simulink model "FMS"  (R2018b)
settings: configuration reference "fms_config" (kept outside this file)
values from neighbouring files (symbols this model uses):
  FMS_EXPORT = Simulink.Parameter(FMS_EXPORT_VALUE)    [fms_model_init.m]
  FMS_PARAM = Simulink.Parameter(FMS_PARAM_VALUE)    [fms_model_init.m]
undefined symbols (not defined in the file or in its folder): actuator_cmd, ax_cmd, ay_cmd, az_cmd, cmd_mask, ControlMode, ctrl_mode, DiscIntNeverNeededParam, ext_state, FMS_Cmd, FMS_CONST, home, mode, p_cmd, phi_cmd, PilotMode, psi_rate_cmd, q_cmd, r_cmd, reset, state, status, theta_cmd, throttle_cmd, timestamp, u_cmd, v_cmd, VehicleState, VehicleStatus, VTOLState, w_cmd, wp_consume, wp_current
libraries: simulink x141, FMT_Model_Lib x120, hdlsllib x13
(part 1 of 12)
settings Model: Creator=jc  LastModifiedBy=zouji
settings ConfigSetRef: SourceLocation=Base Workspace

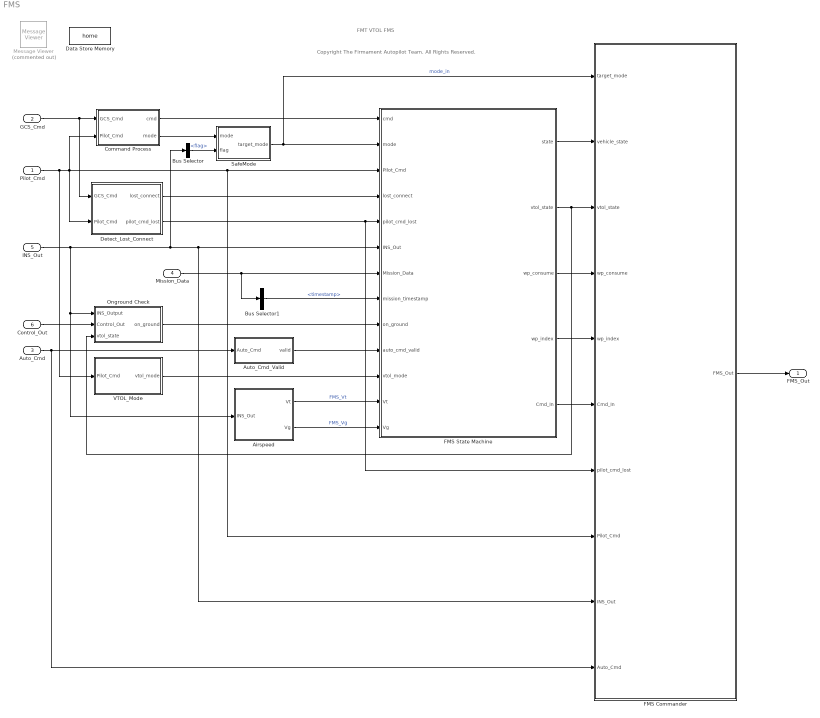
== system FMS ==
  note: Copyright The Firmament Autopilot Team. All Rights Reserved.
  note: FMT VTOL FMS
  Pilot_Cmd : Inport  OutDataTypeStr=Bus: Pilot_Cmd_Bus
  GCS_Cmd : Inport  Port=2  OutDataTypeStr=Bus: GCS_Cmd_Bus
  Auto_Cmd : Inport  Port=3  OutDataTypeStr=Bus: Auto_Cmd_Bus
  Mission_Data : Inport  Port=4  OutDataTypeStr=Bus: Mission_Data_Bus  BusOutputAsStruct=on
  INS_Out : Inport  Port=5  OutDataTypeStr=Bus: INS_Out_Bus
  Control_Out : Inport  Port=6  OutDataTypeStr=Bus: Control_Out_Bus
  Airspeed : Subsystem
  Auto_Cmd_Valid : Subsystem
  Bus Selector : BusSelector  OutputSignals=flag
  Bus Selector1 : BusSelector  OutputSignals=timestamp
  Command Process : Subsystem
  Data Store Memory : DataStoreMemory  DataStoreName=home  ReadBeforeWriteMsg=warning  WriteAfterWriteMsg=warning  WriteAfterReadMsg=warning  ShowAdditionalParam=off  OutDataTypeStr=single  Dimensions=4
  Detect_Lost_Connect : Subsystem
  FMS Commander : Subsystem  TreatAsAtomicUnit=on
  FMS State Machine : Stateflow chart  TreatAsAtomicUnit=on
  Message Viewer : MessageViewer  Commented=on  SavedRootId=#
  Onground Check : Subsystem
  SafeMode : Stateflow chart  TreatAsAtomicUnit=on
  VTOL_Mode : Subsystem
  FMS_Out : Outport  OutDataTypeStr=Bus: FMS_Out_Bus
  wires:
  Control_Out/1 -> Onground Check/2(Control_Out)
  Command Process/1(cmd) -> FMS State Machine/1(cmd)
  FMS State Machine/5(Cmd_In) -> FMS Commander/6(Cmd_In)
  Pilot_Cmd/1 -> VTOL_Mode/1(Pilot_Cmd), Detect_Lost_Connect/2(Pilot_Cmd), FMS Commander/8(Pilot_Cmd), FMS State Machine/3(Pilot_Cmd), Command Process/2(Pilot_Cmd)
  INS_Out/1 -> Airspeed/1(INS_Out), Onground Check/1(INS_Output), Bus Selector/1, FMS Commander/9(INS_Out), FMS State Machine/6(INS_Out)
  Command Process/2(mode) -> SafeMode/1(mode)
  FMS Commander/1(FMS_Out) -> FMS_Out/1
  Onground Check/1(on_ground) -> FMS State Machine/9(on_ground)
  Bus Selector/1 -> SafeMode/2(flag)  "<flag>"
  GCS_Cmd/1 -> Detect_Lost_Connect/1(GCS_Cmd), Command Process/1(GCS_Cmd)
  SafeMode/1(target_mode) -> FMS Commander/1(target_mode), FMS State Machine/2(mode)  "mode_in"
  FMS State Machine/1(state) -> FMS Commander/2(vehicle_state)
  Mission_Data/1 -> Bus Selector1/1, FMS State Machine/7(Mission_Data)
  FMS State Machine/3(wp_consume) -> FMS Commander/4(wp_consume)
  Bus Selector1/1 -> FMS State Machine/8(mission_timestamp)  "<timestamp>"
  FMS State Machine/4(wp_index) -> FMS Commander/5(wp_index)
  Auto_Cmd/1 -> Auto_Cmd_Valid/1(Auto_Cmd), FMS Commander/10(Auto_Cmd)
  Auto_Cmd_Valid/1(valid) -> FMS State Machine/10(auto_cmd_valid)
  Detect_Lost_Connect/1(lost_connect) -> FMS State Machine/4(lost_connect)
  Detect_Lost_Connect/2(pilot_cmd_lost) -> FMS State Machine/5(pilot_cmd_lost), FMS Commander/7(pilot_cmd_lost)
  Airspeed/2(Vg) -> FMS State Machine/13(Vg)  "FMS_Vg"
  Airspeed/1(Vt) -> FMS State Machine/12(Vt)  "FMS_Vt"
  VTOL_Mode/1(vtol_mode) -> FMS State Machine/11(vtol_mode)
  FMS State Machine/2(vtol_state) -> Onground Check/3(vtol_state), FMS Commander/3(vtol_state)

== system FMS/Airspeed ==
  note: If airspeed is invalid, use ground speed
  INS_Out : Inport
  Add : Sum
  Bitwise AND : simulink/Logic and Bit Operations/Bitwise Operator  logicop=AND  UseBitMask=on  BitMask=bin2dec('1000000000')  BitMaskRealWorld=Stored Integer
  Bus Selector1 : BusSelector  OutputSignals=vn,ve
  Bus Selector2 : BusSelector  OutputSignals=flag
  Bus Selector3 : BusSelector  OutputSignals=airspeed
  First Order LPF1 : FMT_Model_Lib/Filter/First Order LPF  fc=20
      settings: SourceProductName=FMT Toolbox
  First Order LPF3 : FMT_Model_Lib/Filter/First Order LPF  fc=10
      settings: SourceProductName=FMT Toolbox
  Fly_Direction : Subsystem
  Fly_Speed : Subsystem
  Multiply : Product
  Saturation1 : Saturate  UpperLimit=100  LowerLimit=0.1
  Sqrt : Sqrt  SaturateOnIntegerOverflow=on
  Square2 : Math  Operator=square  SaturateOnIntegerOverflow=on
  Square3 : Math  Operator=square  SaturateOnIntegerOverflow=on
  Switch : Switch  Criteria=u2 > Threshold
  Vt : Outport
  Vg : Outport  Port=2
  wires:
  Square3/1 -> Add/2
  Sqrt/1 -> Multiply/2
  Bus Selector1/1 -> Square2/1  "<vn>"
  Fly_Direction/1(sign) -> Multiply/1
  Add/1 -> Sqrt/1
  Square2/1 -> Add/1
  Bus Selector1/2 -> Square3/1  "<ve>"
  Multiply/1 -> First Order LPF1/1  "Vg"
  Switch/1 -> Saturation1/1
  Saturation1/1 -> First Order LPF3/1
  INS_Out/1 -> Fly_Direction/1(INS_Out), Bus Selector1/1, Fly_Speed/1(INS_Out), Bus Selector2/1, Bus Selector3/1
  Bitwise AND/1 -> Switch/2
  Bus Selector2/1 -> Bitwise AND/1  "<flag>"
  Bus Selector3/1 -> Switch/1  "<airspeed>"
  First Order LPF1/1 -> Vg/1
  First Order LPF3/1 -> Vt/1
  Fly_Speed/1(speed) -> Switch/3

== system FMS/Auto_Cmd_Valid ==
  Auto_Cmd : Inport
  Bus Selector1 : BusSelector  OutputSignals=frame
  Bus Selector2 : BusSelector  OutputSignals=timestamp
  Compare To Constant4 : simulink/Logic and Bit Operations/Compare To Constant  relop=<  const=1000  OutDataTypeStr=boolean
  Constant : Constant  Value=FMS_EXPORT.period  OutDataTypeStr=single
  Detect Change : simulink/Logic and Bit Operations/Detect Change  vinit=0  OutDataTypeStr=boolean
  Discrete-Time Integrator : DiscreteIntegrator  IntegratorMethod=Accumulation: Forward Euler  ExternalReset=sampled level  SampleTime=-1  OutDataTypeStr=uint32  SaturateOnIntegerOverflow=on  ICPrevOutput=DiscIntNeverNeededParam  ICPrevScaledInput=DiscIntNeverNeededParam
  Ever_Valid : Subsystem
  Interval Test : simulink/Logic and Bit Operations/Interval Test  IntervalClosedRight=on  uplimit=2  IntervalClosedLeft=on  lowlimit=0  OutDataTypeStr=boolean
  Logical Operator : Logic  Inputs=3  AllPortsSameDT=off  OutDataTypeStr=boolean
  valid : Outport
  wires:
  Constant/1 -> Discrete-Time Integrator/1
  Detect Change/1 -> Ever_Valid/1(in), Discrete-Time Integrator/2
  Discrete-Time Integrator/1 -> Compare To Constant4/1
  Auto_Cmd/1 -> Bus Selector1/1, Bus Selector2/1
  Compare To Constant4/1 -> Logical Operator/1
  Ever_Valid/1(out) -> Logical Operator/2
  Logical Operator/1 -> valid/1
  Bus Selector2/1 -> Detect Change/1  "<timestamp>"
  Bus Selector1/1 -> Interval Test/1  "<frame>"
  Interval Test/1 -> Logical Operator/3

== system FMS/Command Process ==
  GCS_Cmd : Inport
  Pilot_Cmd : Inport  Port=2
  Check Valid : Subsystem
  Command PreProcess : Subsystem
  Mode PreProcess : Subsystem
  cmd : Outport
  mode : Outport  Port=2
  wires:
  GCS_Cmd/1 -> Mode PreProcess/2(GCS_Cmd), Command PreProcess/1(gcs_cmd)
  Pilot_Cmd/1 -> Command PreProcess/2(pilot_cmd), Check Valid/1(Pilot_Cmd), Mode PreProcess/3(Pilot_Cmd)
  Command PreProcess/1(cmd_1) -> cmd/1  "fms_cmd"
  Check Valid/1(pilot_cmd_valid) -> Mode PreProcess/1(pilot_cmd_valid)
  Mode PreProcess/1(mode) -> mode/1  "fms_mode"

== system FMS/Detect_Lost_Connect ==
  GCS_Cmd : Inport
  Pilot_Cmd : Inport  Port=2
  Bus Selector : BusSelector  OutputSignals=timestamp
  Bus Selector1 : BusSelector  OutputSignals=timestamp
  Constant : Constant  Value=FMS_CONST.dt  OutDataTypeStr=single
  Constant1 : Constant  Value=FMS_PARAM.LOST_RETURN_EN
  Detect Change : simulink/Logic and Bit Operations/Detect Change  vinit=0  OutDataTypeStr=boolean
  Detect Change1 : simulink/Logic and Bit Operations/Detect Change  vinit=0  OutDataTypeStr=boolean
  Discrete-Time Integrator : DiscreteIntegrator  IntegratorMethod=Accumulation: Forward Euler  ExternalReset=sampled level  SampleTime=-1  OutDataTypeStr=single  SaturateOnIntegerOverflow=on  LimitOutput=on  UpperSaturationLimit=65535  LowerSaturationLimit=0  ICPrevOutput=DiscIntNeverNeededParam  ICPrevScaledInput=DiscIntNeverNeededParam
  Discrete-Time Integrator1 : DiscreteIntegrator  IntegratorMethod=Accumulation: Forward Euler  ExternalReset=sampled level  SampleTime=-1  OutDataTypeStr=single  SaturateOnIntegerOverflow=on  LimitOutput=on  UpperSaturationLimit=65535  LowerSaturationLimit=0  ICPrevOutput=DiscIntNeverNeededParam  ICPrevScaledInput=DiscIntNeverNeededParam
  Logical Operator : Logic  Operator=OR  Inputs=3  AllPortsSameDT=off  OutDataTypeStr=boolean
  Logical Operator1 : Logic  Operator=NOT  AllPortsSameDT=off  OutDataTypeStr=boolean
  Logical Operator2 : Logic  AllPortsSameDT=off  OutDataTypeStr=boolean
  timeout1_s : simulink/Logic and Bit Operations/Compare To Constant  relop=>=  const=FMS_PARAM.LOST_RETURN_TIME  OutDataTypeStr=boolean
  timeout2_s : simulink/Logic and Bit Operations/Compare To Constant  relop=>=  const=1  OutDataTypeStr=boolean
  lost_connect : Outport
  pilot_cmd_lost : Outport  Port=2
  wires:
  Constant/1 -> Discrete-Time Integrator1/1, Discrete-Time Integrator/1
  Discrete-Time Integrator/1 -> timeout1_s/1
  GCS_Cmd/1 -> Bus Selector/1
  Pilot_Cmd/1 -> Bus Selector1/1
  Bus Selector/1 -> Detect Change/1  "<timestamp>"
  Bus Selector1/1 -> Detect Change1/1  "<timestamp>"
  Detect Change/1 -> Logical Operator/1
  Detect Change1/1 -> Discrete-Time Integrator1/2, Logical Operator/2
  Constant1/1 -> Logical Operator2/2, Logical Operator1/1
  Logical Operator1/1 -> Logical Operator/3
  Logical Operator/1 -> Discrete-Time Integrator/2
  Logical Operator2/1 -> lost_connect/1
  timeout1_s/1 -> Logical Operator2/1
  Discrete-Time Integrator1/1 -> timeout2_s/1
  timeout2_s/1 -> pilot_cmd_lost/1

== system FMS/FMS Commander ==
  target_mode : Inport
  vehicle_state : Inport  Port=2
  vtol_state : Inport  Port=3
  wp_consume : Inport  Port=4
  wp_index : Inport  Port=5
  Cmd_In : Inport  Port=6
  pilot_cmd_lost : Inport  Port=7
  Pilot_Cmd : Inport  Port=8
  INS_Out : Inport  Port=9
  Auto_Cmd : Inport  Port=10
  Commander : Subsystem
  FMS_Input : Subsystem  TreatAsAtomicUnit=on
  FMS_Out : Outport
  wires:
  target_mode/1 -> Commander/1(target_mode)
  FMS_Input/1(FMS_In) -> Commander/2(FMS_In)  "FMS_In"
  Commander/1(FMS_Out) -> FMS_Out/1
  vehicle_state/1 -> FMS_Input/1(state)
  wp_consume/1 -> FMS_Input/3(wp_consume)
  wp_index/1 -> FMS_Input/4(wp_index)
  Cmd_In/1 -> FMS_Input/5(Cmd_In)
  Pilot_Cmd/1 -> FMS_Input/7(Pilot_Cmd)
  INS_Out/1 -> FMS_Input/8(INS_Out)
  Auto_Cmd/1 -> FMS_Input/9(Auto_Cmd)
  pilot_cmd_lost/1 -> FMS_Input/6(pilot_cmd_lost)
  vtol_state/1 -> FMS_Input/2(vtol_state)

== system FMS/FMS State Machine/VTOL_State.EndStall ==
  Airspeed : Inport  OutDataTypeStr=single  PortDimensions=1
  f : TriggerPort  TriggerType=function-call  VariantControl=(inherit)  StatesWhenEnabling=reset
      settings: CopyFcn=Stateflow.SLINSF.SimulinkMan.removeBlockPreDeleteFcn  PreDeleteFcn=Stateflow.SLINSF.SimulinkMan.unsafePredeleteFcn
  Constant1 : Constant  Value=FMS_PARAM.FW_SPEED_MIN
  Relational Operator1 : RelationalOperator  OutDataTypeStr=boolean  RndMeth=Simplest
  res : Outport
  wires:
  Airspeed/1 -> Relational Operator1/1
  Constant1/1 -> Relational Operator1/2
  Relational Operator1/1 -> res/1

== system FMS/FMS State Machine/VTOL_State.ForwardTransCplt ==
  Airspeed : Inport  OutDataTypeStr=single  PortDimensions=1
  f : TriggerPort  TriggerType=function-call  VariantControl=(inherit)  StatesWhenEnabling=reset
      settings: CopyFcn=Stateflow.SLINSF.SimulinkMan.removeBlockPreDeleteFcn  PreDeleteFcn=Stateflow.SLINSF.SimulinkMan.unsafePredeleteFcn
  Constant : Constant  Value=FMS_PARAM.FW_SPEED_MIN
  Relational Operator : RelationalOperator  OutDataTypeStr=boolean  RndMeth=Simplest
  cplt : Outport
  wires:
  Airspeed/1 -> Relational Operator/1
  Constant/1 -> Relational Operator/2
  Relational Operator/1 -> cplt/1

== system FMS/FMS State Machine/VTOL_State.IsPosValid ==
  flag : Inport  OutDataTypeStr=uint32  PortDimensions=1
  f : TriggerPort  TriggerType=function-call  VariantControl=(inherit)  StatesWhenEnabling=reset
      settings: CopyFcn=Stateflow.SLINSF.SimulinkMan.removeBlockPreDeleteFcn  PreDeleteFcn=Stateflow.SLINSF.SimulinkMan.unsafePredeleteFcn
  Bitwise AND : simulink/Logic and Bit Operations/Bitwise Operator  logicop=AND  UseBitMask=on  BitMask=bin2dec('11010100')  BitMaskRealWorld=Stored Integer
  Compare To Constant : simulink/Logic and Bit Operations/Compare To Constant  relop===  const=bin2dec('11010100')  OutDataTypeStr=boolean
  valid : Outport
  wires:
  flag/1 -> Bitwise AND/1
  Bitwise AND/1 -> Compare To Constant/1
  Compare To Constant/1 -> valid/1

== system FMS/FMS State Machine/VTOL_State.IsStall ==
  Airspeed : Inport  OutDataTypeStr=single  PortDimensions=1
  f : TriggerPort  TriggerType=function-call  VariantControl=(inherit)  StatesWhenEnabling=reset
      settings: CopyFcn=Stateflow.SLINSF.SimulinkMan.removeBlockPreDeleteFcn  PreDeleteFcn=Stateflow.SLINSF.SimulinkMan.unsafePredeleteFcn
  Constant1 : Constant  Value=FMS_PARAM.FW_STALL_SPEED
  Relational Operator1 : RelationalOperator  Operator=<=  OutDataTypeStr=boolean  RndMeth=Simplest
  res : Outport
  wires:
  Airspeed/1 -> Relational Operator1/1
  Constant1/1 -> Relational Operator1/2
  Relational Operator1/1 -> res/1

== system FMS/FMS State Machine/Vehicle.AcceptRadius ==
  state : Inport  OutDataTypeStr=Enum: VTOLState  PortDimensions=1
  f : TriggerPort  TriggerType=function-call  VariantControl=(inherit)  StatesWhenEnabling=reset
      settings: CopyFcn=Stateflow.SLINSF.SimulinkMan.removeBlockPreDeleteFcn  PreDeleteFcn=Stateflow.SLINSF.SimulinkMan.unsafePredeleteFcn
  Compare To Constant : simulink/Logic and Bit Operations/Compare To Constant  relop===  const=VTOLState.Multicopter  OutDataTypeStr=boolean
  FW_ACCEPT_R : Constant  Value=FMS_PARAM.FW_ACCEPT_R
  MC_ACCEPT_R : Constant  Value=FMS_PARAM.MC_ACCEPT_R
  Switch : Switch  Criteria=u2 > Threshold
  radius : Outport
  wires:
  Compare To Constant/1 -> Switch/2
  FW_ACCEPT_R/1 -> Switch/3
  MC_ACCEPT_R/1 -> Switch/1
  Switch/1 -> radius/1
  state/1 -> Compare To Constant/1

== system FMS/FMS State Machine/Vehicle.Arm.Auto.Mission.LLA2FLAT ==
  lla : Inport  OutDataTypeStr=double  PortDimensions=[1 3]
  llo : Inport  Port=2  OutDataTypeStr=double  Unit=deg  PortDimensions=[1 2]
  href : Inport  Port=3  OutDataTypeStr=double  Unit=m  PortDimensions=1
  psio : Inport  Port=4  OutDataTypeStr=double  Unit=deg  PortDimensions=1
  f : TriggerPort  TriggerType=function-call  VariantControl=(inherit)
      settings: CopyFcn=Stateflow.SLINSF.SimulinkMan.removeBlockPreDeleteFcn  PreDeleteFcn=Stateflow.SLINSF.SimulinkMan.unsafePredeleteFcn
  Data Type Conversion : DataTypeConversion  OutDataTypeStr=single
  LLA2FLAT : FMT_Model_Lib/Transformation/LLA2FLAT
      settings: SourceProductName=FMT Toolbox
  Signal Conversion : SignalConversion  OverrideOpt=off
  pos : Outport
  wires:
  LLA2FLAT/1 -> Signal Conversion/1
  lla/1 -> LLA2FLAT/1
  llo/1 -> LLA2FLAT/2
  href/1 -> LLA2FLAT/3
  psio/1 -> LLA2FLAT/4
  Signal Conversion/1 -> Data Type Conversion/1
  Data Type Conversion/1 -> pos/1

== system FMS/FMS State Machine/Vehicle.HeadingErr ==
  psi_cmd : Inport  OutDataTypeStr=single  PortDimensions=1
  psi_est : Inport  Port=2  OutDataTypeStr=single  Unit=deg  PortDimensions=1
  f : TriggerPort  TriggerType=function-call  VariantControl=(inherit)
      settings: CopyFcn=Stateflow.SLINSF.SimulinkMan.removeBlockPreDeleteFcn  PreDeleteFcn=Stateflow.SLINSF.SimulinkMan.unsafePredeleteFcn
  Sum : Sum  Inputs=|+-
  psi_saturation : Subsystem
  err : Outport
  wires:
  psi_saturation/1(psi_rad) -> err/1
  psi_est/1 -> Sum/2
  psi_cmd/1 -> Sum/1
  Sum/1 -> psi_saturation/1(psi_in)

== system FMS/FMS State Machine/Vehicle.PrepTakeoff ==
  xy_R : Inport  OutDataTypeStr=single  PortDimensions=2
  f : TriggerPort  TriggerType=function-call  VariantControl=(inherit)  StatesWhenEnabling=reset
      settings: CopyFcn=Stateflow.SLINSF.SimulinkMan.removeBlockPreDeleteFcn  PreDeleteFcn=Stateflow.SLINSF.SimulinkMan.unsafePredeleteFcn
  Constant : Constant  Value=FMS_PARAM.TAKEOFF_H
  Mux : Mux  Inputs=2
  Reshape : Reshape  OutputDimensionality=Column vector (2-D)
  sp_takeoff : Outport
  wires:
  Reshape/1 -> sp_takeoff/1
  xy_R/1 -> Mux/1
  Mux/1 -> Reshape/1
  Constant/1 -> Mux/2

== system FMS/FMS State Machine/Vehicle.StickMoved ==
  stick_val : Inport  OutDataTypeStr=double  PortDimensions=4
  pilot_cmd : Inport  Port=2  OutDataTypeStr=Bus: Pilot_Cmd_Bus  PortDimensions=1
  f : TriggerPort  TriggerType=function-call  VariantControl=(inherit)
      settings: CopyFcn=Stateflow.SLINSF.SimulinkMan.removeBlockPreDeleteFcn  PreDeleteFcn=Stateflow.SLINSF.SimulinkMan.unsafePredeleteFcn
  Abs : Abs
  Bus Selector : BusSelector  OutputSignals=stick_yaw,stick_throttle,stick_roll,stick_pitch
  Compare To Constant : simulink/Logic and Bit Operations/Compare To Constant  relop=>=  const=0.1  OutDataTypeStr=boolean
  Max : MinMax  Function=max
  Mux : Mux
  Sum : Sum  Inputs=|+-
  moved : Outport
  wires:
  pilot_cmd/1 -> Bus Selector/1
  Bus Selector/1 -> Mux/1  "<stick_yaw>"
  Bus Selector/2 -> Mux/2  "<stick_throttle>"
  Bus Selector/3 -> Mux/3  "<stick_roll>"
  Bus Selector/4 -> Mux/4  "<stick_pitch>"
  stick_val/1 -> Sum/1
  Mux/1 -> Sum/2
  Sum/1 -> Abs/1
  Abs/1 -> Max/1
  Max/1 -> Compare To Constant/1
  Compare To Constant/1 -> moved/1

== system FMS/FMS State Machine/Vehicle.WaypointAngle ==
  start : Inport  OutDataTypeStr=single  PortDimensions=[3 1]
  end : Inport  Port=2  OutDataTypeStr=single  PortDimensions=[3 1]
  f : TriggerPort  TriggerType=function-call  VariantControl=(inherit)
      settings: CopyFcn=Stateflow.SLINSF.SimulinkMan.removeBlockPreDeleteFcn  PreDeleteFcn=Stateflow.SLINSF.SimulinkMan.unsafePredeleteFcn
  Bias : Bias  Bias=2*pi
  Included Angle : Subsystem
  North : Constant  Value=[1 0]  OutDataTypeStr=single
  Selector : Selector  InputPortWidth=3  IndexOptions=Index vector (dialog)  Indices=[1 2]  OutputSizes=1
  Selector1 : Selector  InputPortWidth=3  IndexOptions=Index vector (dialog)  Indices=[1 2]  OutputSizes=1
  Sum : Sum  Inputs=|+-
  Switch : Switch
  angle : Outport
  wires:
  Selector/1 -> Sum/1
  Selector1/1 -> Sum/2
  North/1 -> Included Angle/1(vec1)
  Sum/1 -> Included Angle/2(vec2)
  Included Angle/1(angle_rad) -> Switch/1, Bias/1, Switch/2
  Switch/1 -> angle/1
  Bias/1 -> Switch/3
  start/1 -> Selector1/1
  end/1 -> Selector/1

== system FMS/Onground Check ==
  INS_Output : Inport
  Control_Out : Inport  Port=2
  vtol_state : Inport  Port=3
  Bus Selector : BusSelector  OutputSignals=quat
  Bus Selector1 : BusSelector  OutputSignals=actuator_cmd
  Bus Selector2 : BusSelector  OutputSignals=phi,theta
  Bus Selector3 : BusSelector  OutputSignals=ax,ay,az
  Compare To Constant : simulink/Logic and Bit Operations/Compare To Constant  relop=>=  const=10000  OutDataTypeStr=boolean
  Compare To Constant1 : simulink/Logic and Bit Operations/Compare To Constant  relop=~=  const=VTOLState.Multicopter  OutDataTypeStr=boolean
  Constant : Constant  Value=4  OutDataTypeStr=uint16
  Constant1 : Constant  Value=FMS_EXPORT.period  OutDataTypeStr=single
  Cos : Trigonometry  Operator=cos
  Cos1 : Trigonometry  Operator=cos
  Delay : Delay  DelayLength=1  InitialCondition=1
  Discrete-Time Integrator : DiscreteIntegrator  IntegratorMethod=Accumulation: Forward Euler  ExternalReset=level  SampleTime=-1  OutDataTypeStr=uint32  SaturateOnIntegerOverflow=on  LimitOutput=on  UpperSaturationLimit=1e6  LowerSaturationLimit=0  ICPrevOutput=DiscIntNeverNeededParam  ICPrevScaledInput=DiscIntNeverNeededParam
  Divide : Product  Inputs=*/
  Divide1 : Product  Inputs=/*
  First Order LPF : FMT_Model_Lib/Filter/First Order LPF  fc=1/(2*pi*0.5)
      settings: SourceProductName=FMT Toolbox
  First Order LPF1 : FMT_Model_Lib/Filter/First Order LPF  fc=1/(2*pi*0.1)
      settings: SourceProductName=FMT Toolbox
  First Order LPF2 : FMT_Model_Lib/Filter/First Order LPF  fc=1/(2*pi*0.1)
      settings: SourceProductName=FMT Toolbox
  Interval Test : simulink/Logic and Bit Operations/Interval Test  IntervalClosedRight=on  uplimit=[0.5, 0.5, -9.806+0.5]  IntervalClosedLeft=on  lowlimit=[-0.5, -0.5, -9.806-0.5]  OutDataTypeStr=boolean
  Land_Lock_Thro : Constant  Value=FMS_PARAM.LAND_LOCK_THRO
  Logical Operator : Logic  Inputs=1  AllPortsSameDT=off  OutDataTypeStr=boolean
  Logical Operator1 : Logic  Inputs=3  AllPortsSameDT=off  OutDataTypeStr=boolean
  Matrix Concatenate3 : Concatenate  NumInputs=3  ConcatenateDimension=2
  Multiply : Product  Multiplication=Matrix(*)
  Multiply1 : Product
  Quaternion To DCM : FMT_Model_Lib/Quaternion/Quaternion To DCM
      settings: SourceProductName=FMT Toolbox
  Relational Operator : RelationalOperator  Operator=<  OutDataTypeStr=boolean  RndMeth=Simplest
  Saturation : Saturate  UpperLimit=1  LowerLimit=0.9
  Selector : Selector  InputPortWidth=16  IndexOptions=Index vector (dialog)  Indices=[1:4]  OutputSizes=1
  Sum of Elements : Sum  Inputs=+
  Transpose : Math  Operator=transpose  SaturateOnIntegerOverflow=on
  on_ground : Outport
  wires:
  Bus Selector3/2 -> Matrix Concatenate3/2  "<ay>"
  Relational Operator/1 -> Logical Operator1/2
  Bus Selector3/3 -> Matrix Concatenate3/3  "<az>"
  Bus Selector1/1 -> Selector/1  "<actuator_cmd>"
  Bus Selector3/1 -> Matrix Concatenate3/1  "<ax>"
  Selector/1 -> Sum of Elements/1
  INS_Output/1 -> Bus Selector2/1, Bus Selector3/1, Bus Selector/1
  Control_Out/1 -> Bus Selector1/1
  Interval Test/1 -> Logical Operator/1
  Sum of Elements/1 -> Divide/1
  Constant/1 -> Divide/2
  First Order LPF/1 -> Interval Test/1
  Divide/1 -> First Order LPF2/1
  First Order LPF2/1 -> Relational Operator/1
  Logical Operator/1 -> Logical Operator1/1
  Logical Operator1/1 -> on_ground/1  "on_ground"
  Bus Selector/1 -> Quaternion To DCM/1  "<quat>"
  Quaternion To DCM/1 -> Transpose/1
  Matrix Concatenate3/1 -> Multiply/2
  Transpose/1 -> Multiply/1
  Multiply/1 -> First Order LPF/1
  Bus Selector2/1 -> Cos/1  "<phi>"
  Bus Selector2/2 -> Cos1/1  "<theta>"
  Cos/1 -> Multiply1/1
  Cos1/1 -> Multiply1/2
  Multiply1/1 -> Saturation/1
  Saturation/1 -> Divide1/1
  Divide1/1 -> First Order LPF1/1
  First Order LPF1/1 -> Relational Operator/2
  Land_Lock_Thro/1 -> Divide1/2
  Constant1/1 -> Discrete-Time Integrator/1
  vtol_state/1 -> Compare To Constant1/1
  Discrete-Time Integrator/1 -> Compare To Constant/1
  Compare To Constant/1 -> Logical Operator1/3
  Delay/1 -> Discrete-Time Integrator/2
  Compare To Constant1/1 -> Delay/1

== system FMS/VTOL_Mode ==
  Pilot_Cmd : Inport
  Bus Selector2 : BusSelector  OutputSignals=cmd_2
  Data Type Conversion : DataTypeConversion  OutDataTypeStr=Enum: VTOLMode
  vtol_mode : Outport
  wires:
  Bus Selector2/1 -> Data Type Conversion/1  "<cmd_2>"
  Pilot_Cmd/1 -> Bus Selector2/1
  Data Type Conversion/1 -> vtol_mode/1

== system FMS/Airspeed/Fly_Direction ==
  INS_Out : Inport
  Bus Selector2 : BusSelector  OutputSignals=vn,ve,vd
  Bus Selector3 : BusSelector  OutputSignals=psi
  Multiply : Product  Multiplication=Matrix(*)
  Mux : Mux  Inputs=3
  Psi To DCM : FMT_Model_Lib/Transformation/Psi To DCM
      settings: SourceProductName=FMT Toolbox
  Selector : Selector  InputPortWidth=3  IndexOptions=Index vector (dialog)  Indices=1  OutputSizes=1
  Sign : Signum
  sign : Outport
  wires:
  Bus Selector3/1 -> Psi To DCM/1  "<psi>"
  Multiply/1 -> Selector/1
  Bus Selector2/3 -> Mux/3  "<vd>"
  INS_Out/1 -> Bus Selector3/1, Bus Selector2/1
  Sign/1 -> sign/1
  Mux/1 -> Multiply/2
  Psi To DCM/1 -> Multiply/1
  Bus Selector2/2 -> Mux/2  "<ve>"
  Bus Selector2/1 -> Mux/1  "<vn>"
  Selector/1 -> Sign/1  "Vu"

== system FMS/Airspeed/Fly_Speed ==
  INS_Out : Inport
  Bus Selector2 : BusSelector  OutputSignals=vn,ve,vd
  Bus Selector3 : BusSelector  OutputSignals=quat
  Multiply : Product  Multiplication=Matrix(*)
  Mux : Mux  Inputs=3
  Quaternion To DCM : FMT_Model_Lib/Quaternion/Quaternion To DCM
      settings: SourceProductName=FMT Toolbox
  Selector : Selector  InputPortWidth=3  IndexOptions=Index vector (dialog)  Indices=1  OutputSizes=1
  speed : Outport
  wires:
  Bus Selector3/1 -> Quaternion To DCM/1  "<quat>"
  Multiply/1 -> Selector/1
  Bus Selector2/3 -> Mux/3  "<vd>"
  INS_Out/1 -> Bus Selector3/1, Bus Selector2/1
  Mux/1 -> Multiply/2
  Quaternion To DCM/1 -> Multiply/1
  Bus Selector2/2 -> Mux/2  "<ve>"
  Bus Selector2/1 -> Mux/1  "<vn>"
  Selector/1 -> speed/1

== system FMS/Auto_Cmd_Valid/Ever_Valid ==
  in : Inport
  Constant1 : Constant  OutDataTypeStr=uint8
  Delay : Delay  DelayLength=1
  Switch : Switch  Criteria=u2 > Threshold
  out : Outport
  wires:
  Constant1/1 -> Switch/1
  Delay/1 -> Switch/3
  in/1 -> Switch/2
  Switch/1 -> out/1, Delay/1

== system FMS/Command Process/Check Valid ==
  Pilot_Cmd : Inport
  Bus Selector1 : BusSelector  OutputSignals=timestamp
  Compare To Constant1 : simulink/Logic and Bit Operations/Compare To Constant  relop=<  const=500  OutDataTypeStr=boolean
  Constant1 : Constant  Value=FMS_EXPORT.period  OutDataTypeStr=single
  Detect Change1 : simulink/Logic and Bit Operations/Detect Change  vinit=0  OutDataTypeStr=boolean
  Discrete-Time Integrator1 : DiscreteIntegrator  IntegratorMethod=Accumulation: Forward Euler  ExternalReset=sampled level  SampleTime=-1  OutDataTypeStr=uint32  SaturateOnIntegerOverflow=on  ICPrevOutput=DiscIntNeverNeededParam  ICPrevScaledInput=DiscIntNeverNeededParam
  pilot_cmd_valid : Outport
  wires:
  Pilot_Cmd/1 -> Bus Selector1/1
  Compare To Constant1/1 -> pilot_cmd_valid/1
  Bus Selector1/1 -> Detect Change1/1  "<timestamp>"
  Constant1/1 -> Discrete-Time Integrator1/1
  Detect Change1/1 -> Discrete-Time Integrator1/2
  Discrete-Time Integrator1/1 -> Compare To Constant1/1

== system FMS/Command Process/Command PreProcess ==
  gcs_cmd : Inport
  pilot_cmd : Inport  Port=2
  Bus Selector : BusSelector  OutputSignals=cmd_1
  Bus Selector1 : BusSelector  OutputSignals=cmd_1
  Bus Selector2 : BusSelector  OutputSignals=param
  Compare To Constant : simulink/Logic and Bit Operations/Compare To Constant  relop===  const=FMS_Cmd.SetHome  OutDataTypeStr=boolean
  Constant1 : Constant  Value=FMS_Cmd.None
  Data Type Conversion1 : DataTypeConversion  OutDataTypeStr=Enum: FMS_Cmd
  Data Type Conversion2 : DataTypeConversion  OutDataTypeStr=Enum: FMS_Cmd
  Detect Change3 : simulink/Logic and Bit Operations/Detect Change  vinit=0  OutDataTypeStr=boolean
  Detect Change4 : simulink/Logic and Bit Operations/Detect Change  vinit=0  OutDataTypeStr=boolean
  Selector : Selector  InputPortWidth=7  IndexOptions=Index vector (dialog)  Indices=[1:4]  OutputSizes=1
  SetHome : Subsystem  TreatAsAtomicUnit=on
  Switch1 : Switch  Criteria=u2 > Threshold
  Switch2 : Switch  Criteria=u2 > Threshold
  cmd_1 : Outport
  wires:
  Bus Selector/1 -> Data Type Conversion1/1, Detect Change4/1  "<cmd_1>"
  pilot_cmd/1 -> Bus Selector1/1
  Switch1/1 -> cmd_1/1
  gcs_cmd/1 -> Bus Selector2/1, Bus Selector/1
  Bus Selector1/1 -> Data Type Conversion2/1, Detect Change3/1  "<cmd_1>"
  Detect Change3/1 -> Switch1/2
  Switch2/1 -> Switch1/3
  Detect Change4/1 -> Switch2/2
  Data Type Conversion2/1 -> Switch1/1
  Data Type Conversion1/1 -> Compare To Constant/1, Switch2/1
  Constant1/1 -> Switch2/3
  Compare To Constant/1 -> SetHome/Trigger
  Bus Selector2/1 -> Selector/1  "<param>"
  Selector/1 -> SetHome/1(home)

== system FMS/Command Process/Mode PreProcess ==
  pilot_cmd_valid : Inport
  GCS_Cmd : Inport  Port=2
  Pilot_Cmd : Inport  Port=3
  Bus Selector1 : BusSelector  OutputSignals=mode
  Bus Selector2 : BusSelector  OutputSignals=mode
  Compare To Zero : simulink/Logic and Bit Operations/Compare To Zero  relop=~=  OutDataTypeStr=boolean
  Compare To Zero1 : simulink/Logic and Bit Operations/Compare To Zero  relop=~=  OutDataTypeStr=boolean
  Data Type Conversion1 : DataTypeConversion  OutDataTypeStr=Enum: PilotMode
  Data Type Conversion2 : DataTypeConversion  OutDataTypeStr=Enum: PilotMode
  Delay : Delay  DelayLength=1  InitialCondition=PilotMode.None
  Detect Change : simulink/Logic and Bit Operations/Detect Change  vinit=0  OutDataTypeStr=boolean
  Logical Operator : Logic  AllPortsSameDT=off  OutDataTypeStr=boolean
  Logical Operator1 : Logic  AllPortsSameDT=off  OutDataTypeStr=boolean
  Switch : Switch  Criteria=u2 > Threshold
  Switch1 : Switch  Criteria=u2 > Threshold
  mode : Outport
  wires:
  Bus Selector2/1 -> Compare To Zero/1, Detect Change/1, Data Type Conversion1/1  "<mode>"
  GCS_Cmd/1 -> Bus Selector2/1
  Pilot_Cmd/1 -> Bus Selector1/1
  Bus Selector1/1 -> Compare To Zero1/1, Data Type Conversion2/1  "<mode>"
  Logical Operator1/1 -> Switch/2
  Data Type Conversion2/1 -> Switch/1
  Switch/1 -> mode/1, Delay/1
  Delay/1 -> Switch1/3
  Compare To Zero/1 -> Logical Operator/2
  Data Type Conversion1/1 -> Switch1/1
  Switch1/1 -> Switch/3
  Detect Change/1 -> Logical Operator/1
  Logical Operator/1 -> Switch1/2
  pilot_cmd_valid/1 -> Logical Operator1/2
  Compare To Zero1/1 -> Logical Operator1/1

== system FMS/FMS Commander/Commander ==
  target_mode : Inport
  FMS_In : Inport  Port=2
  Arm : Subsystem  TreatAsAtomicUnit=on
  Bus Selector1 : BusSelector  OutputSignals=vehicle_state
  Bus_Constructor : Subsystem
  Disarm : Subsystem  TreatAsAtomicUnit=on
  FMS_In1 : InportShadow  Port=2
  FMS_In2 : InportShadow  Port=2
  Merge : Merge  Inputs=3
  Standby : Subsystem  TreatAsAtomicUnit=on
  Switch Case : SwitchCase  CaseConditions={[VehicleState.Disarm,VehicleState.None], VehicleState.Standby}
  FMS_Out : Outport
  wires:
  Switch Case/3 -> Arm/Action
  Bus Selector1/1 -> Switch Case/1  "<vehicle_state>"
  FMS_In/1 -> Bus Selector1/1
  Standby/1(FMS_Out) -> Merge/2
  Arm/1(FMS_Out) -> Merge/3
  Switch Case/2 -> Standby/Action
  Switch Case/1 -> Disarm/Action
  Disarm/1(FMS_Out) -> Merge/1
  Merge/1 -> Bus_Constructor/1(Bus_In)
  target_mode/1 -> Bus_Constructor/2(target_mode)
  FMS_In2/1 -> Bus_Constructor/3(FMS_In)
  Bus_Constructor/1(FMS_Out) -> FMS_Out/1
  FMS_In1/1 -> Arm/1(FMS_In)

== system FMS/FMS Commander/FMS_Input ==
  state : Inport
  vtol_state : Inport  Port=2
  wp_consume : Inport  Port=3
  wp_index : Inport  Port=4
  Cmd_In : Inport  Port=5
  pilot_cmd_lost : Inport  Port=6
  Pilot_Cmd : Inport  Port=7
  INS_Out : Inport  Port=8
  Auto_Cmd : Inport  Port=9
  Bus Creator : BusCreator  Inputs=9
  Signal Copy{,1..8} (9 alike) : SignalConversion  OverrideOpt=off
  FMS_In : Outport
  wires:
  Bus Creator/1 -> FMS_In/1
  Pilot_Cmd/1 -> Signal Copy2/1
  Auto_Cmd/1 -> Signal Copy/1
  INS_Out/1 -> Signal Copy1/1
  Signal Copy2/1 -> Bus Creator/7  "Pilot_Cmd"
  Signal Copy/1 -> Bus Creator/9  "Auto_Cmd"
  Signal Copy1/1 -> Bus Creator/8  "INS_Out"
  Cmd_In/1 -> Signal Copy3/1
  Signal Copy3/1 -> Bus Creator/5  "Cmd_In"
  wp_index/1 -> Signal Copy5/1
  Signal Copy5/1 -> Bus Creator/4  "wp_index"
  wp_consume/1 -> Signal Copy4/1
  Signal Copy4/1 -> Bus Creator/3  "wp_consume"
  state/1 -> Signal Copy6/1
  Signal Copy6/1 -> Bus Creator/1  "vehicle_state"
  pilot_cmd_lost/1 -> Signal Copy7/1
  Signal Copy7/1 -> Bus Creator/6  "pilot_cmd_lost"
  vtol_state/1 -> Signal Copy8/1
  Signal Copy8/1 -> Bus Creator/2  "vtol_state"

== system FMS/FMS State Machine/Vehicle.HeadingErr/psi_saturation ==
  psi_in : Inport
  Abs : Abs
  Add : Sum  Inputs=-+
  Compare To Constant : simulink/Logic and Bit Operations/Compare To Constant  relop=>  const=pi  OutDataTypeStr=boolean
  Constant : Constant  Value=2*pi  OutDataTypeStr=single
  Constant1 : Constant  Value=2*pi  OutDataTypeStr=single
  Multiply : Product
  Rem : Math  Operator=rem  SaturateOnIntegerOverflow=on
  Sign : Signum
  Switch : Switch  Criteria=u2 > Threshold
  psi_rad : Outport
  wires:
  Rem/1 -> Sign/1, Add/2, Switch/3, Abs/1
  Abs/1 -> Compare To Constant/1
  Compare To Constant/1 -> Switch/2
  Add/1 -> Switch/1
  Multiply/1 -> Add/1
  Constant/1 -> Multiply/1
  Sign/1 -> Multiply/2
  Switch/1 -> psi_rad/1
  psi_in/1 -> Rem/1
  Constant1/1 -> Rem/2

== system FMS/FMS State Machine/Vehicle.WaypointAngle/Included Angle ==
  vec1 : Inport
  vec2 : Inport  Port=2
  2D Cross Product : FMT_Model_Lib/Math/2D Cross Product
      settings: SourceProductName=FMT Toolbox
  Acos : Trigonometry  Operator=acos
  Constant4 : Constant  OutDataTypeStr=single
  Demux : Demux  Outputs=2
  Demux1 : Demux  Outputs=2
  Dot Product : DotProduct  InputSameDT=on  OutDataTypeStr=Inherit: Inherit via internal rule
  Multiply : Product
  Mux : Mux  Inputs=2
  Mux1 : Mux  Inputs=2
  Sign1 : Signum
  Switch2 : Switch  Criteria=u2 ~= 0
  Vector Normalize : FMT_Model_Lib/Math/Vector Normalize
      settings: SourceProductName=FMT Toolbox
  Vector Normalize1 : FMT_Model_Lib/Math/Vector Normalize
      settings: SourceProductName=FMT Toolbox
  angle_rad : Outport
  wires:
  Switch2/1 -> Multiply/2
  Acos/1 -> Multiply/1
  Mux/1 -> Vector Normalize1/1
  vec2/1 -> Demux/1
  Constant4/1 -> Switch2/3
  Demux/1 -> Mux/2
  vec1/1 -> Demux1/1
  Multiply/1 -> angle_rad/1
  2D Cross Product/1 -> Sign1/1
  Vector Normalize/1 -> 2D Cross Product/2, Dot Product/1
  Demux/2 -> Mux/1
  Vector Normalize1/1 -> 2D Cross Product/1, Dot Product/2
  Sign1/1 -> Switch2/2, Switch2/1
  Demux1/2 -> Mux1/1
  Mux1/1 -> Vector Normalize/1
  Demux1/1 -> Mux1/2
  Dot Product/1 -> Acos/1

== system FMS/Command Process/Command PreProcess/SetHome ==
  home : Inport
  Trigger : TriggerPort  VariantControl=Variant
  Data Store Write : DataStoreWrite  DataStoreName=home
  wires:
  home/1 -> Data Store Write/1

== system FMS/FMS Commander/Commander/Arm ==
  In Bus Element{1..4} (4 alike) : Inport  PortName=FMS_In
  Action Port : ActionPort  InitializeStates=reset  ActionType=default
  BackwardTrans_Mode : Subsystem  TreatAsAtomicUnit=on
  Bus Selector : BusSelector  OutputSignals=vtol_state
  FW_Mode : Subsystem  TreatAsAtomicUnit=on
  MC_Mode : Subsystem  TreatAsAtomicUnit=on
  Merge : Merge  Inputs=3
  Switch Case : SwitchCase  CaseConditions={[VTOLState.Fixwing,VTOLState.ForwardTrans,VTOLState.Stall], VTOLState.BackwardTrans}
  FMS_Out : Outport
  wires:
  Merge/1 -> FMS_Out/1
  In Bus Element2/1 -> Bus Selector/1
  Bus Selector/1 -> Switch Case/1  "<vtol_state>"
  In Bus Element1/1 -> MC_Mode/1(FMS_In)
  In Bus Element3/1 -> FW_Mode/1(FMS_In)
  Switch Case/1 -> FW_Mode/Action
  Switch Case/3 -> MC_Mode/Action
  Switch Case/2 -> BackwardTrans_Mode/Action
  BackwardTrans_Mode/1(FMS_Out) -> Merge/2
  FW_Mode/1(FMS_Out) -> Merge/1
  MC_Mode/1(FMS_Out) -> Merge/3
  In Bus Element4/1 -> BackwardTrans_Mode/1(FMS_In)

== system FMS/FMS Commander/Commander/Bus_Constructor ==
  Bus_In : Inport
  target_mode : Inport  Port=2
  FMS_In : Inport  Port=3
  Bus Assignment : BusAssignment  AssignedSignals=timestamp,mode,ext_state,wp_consume,wp_current,home
  Bus Selector : BusSelector  OutputSignals=vtol_state,wp_consume,wp_index
  Constant : Constant  OutDataTypeStr=uint8
  Data Store Read : DataStoreRead  DataStoreName=home
  Data Type Conversion : DataTypeConversion
  Data Type Conversion2 : DataTypeConversion  OutDataTypeStr=uint8
  Sum : Sum  Inputs=-+|
  timestamp : Subsystem  mask{sample_time=FMS_EXPORT.period}
      mask prompts: sample_time "sample time (ms)"
  FMS_Out : Outport
  wires:
  target_mode/1 -> Data Type Conversion/1
  Bus_In/1 -> Bus Assignment/1
  Bus Assignment/1 -> FMS_Out/1
  FMS_In/1 -> Bus Selector/1
  Bus Selector/3 -> Sum/2  "<wp_index>"
  Constant/1 -> Sum/1
  Data Store Read/1 -> Bus Assignment/7
  Sum/1 -> Bus Assignment/6
  Bus Selector/2 -> Bus Assignment/5  "<wp_consume>"
  Data Type Conversion/1 -> Bus Assignment/3
  timestamp/1(timestamp_ms) -> Bus Assignment/2
  Bus Selector/1 -> Data Type Conversion2/1  "<vtol_state>"
  Data Type Conversion2/1 -> Bus Assignment/4

== system FMS/FMS Commander/Commander/Disarm ==
  Action Port : ActionPort  InitializeStates=reset  ActionType=case
  Bus Assignment : BusAssignment  AssignedSignals=reset,status,state
  Constant : Constant  Value=0  OutDataTypeStr=Bus: FMS_Out_Bus
  Constant1 : Constant  Value=VehicleStatus.Disarm
  Constant2 : Constant  OutDataTypeStr=Inherit: Inherit via back propagation
  Constant5 : Constant  Value=VehicleState.Disarm
  Data Type Conversion : DataTypeConversion
  Data Type Conversion1 : DataTypeConversion
  FMS_Out : Outport
  wires:
  Constant1/1 -> Data Type Conversion/1
  Constant2/1 -> Bus Assignment/2
  Bus Assignment/1 -> FMS_Out/1
  Constant/1 -> Bus Assignment/1
  Constant5/1 -> Data Type Conversion1/1
  Data Type Conversion/1 -> Bus Assignment/3
  Data Type Conversion1/1 -> Bus Assignment/4

== system FMS/FMS Commander/Commander/Standby ==
  Action Port : ActionPort  InitializeStates=reset  ActionType=case
  Bus Assignment : BusAssignment  AssignedSignals=reset,status,state
  Constant : Constant  Value=0  OutDataTypeStr=Bus: FMS_Out_Bus
  Constant1 : Constant  Value=VehicleStatus.Standby
  Constant2 : Constant  OutDataTypeStr=Inherit: Inherit via back propagation
  Constant5 : Constant  Value=VehicleState.Standby
  Data Type Conversion1 : DataTypeConversion
  Data Type Conversion2 : DataTypeConversion
  FMS_Out : Outport
  wires:
  Constant/1 -> Bus Assignment/1
  Bus Assignment/1 -> FMS_Out/1
  Constant2/1 -> Bus Assignment/2
  Constant1/1 -> Data Type Conversion2/1
  Constant5/1 -> Data Type Conversion1/1
  Data Type Conversion2/1 -> Bus Assignment/3
  Data Type Conversion1/1 -> Bus Assignment/4

== system FMS/FMS Commander/Commander/Arm/BackwardTrans_Mode ==
  FMS_In : Inport
  Action Port : ActionPort  InitializeStates=reset  ActionType=case
      settings: CopyFcn=Stateflow.SLINSF.SimulinkMan.removeBlockPreDeleteFcn
  Bus Assignment : BusAssignment  AssignedSignals=status,state,ctrl_mode,u_cmd,v_cmd,w_cmd,psi_rate_cmd,ay_cmd
  Constant : Constant  Value=0  OutDataTypeStr=Bus: FMS_Out_Bus
  Constant1 : Constant  Value=VehicleState.Hold
  Constant2 : Constant  Value=ControlMode.POSCTL
  Constant3 : Constant  Value=0  OutDataTypeStr=single
  Constant5 : Constant  Value=VehicleStatus.Arm
  Data Type Conversion1 : DataTypeConversion
  Data Type Conversion2 : DataTypeConversion
  Data Type Conversion3 : DataTypeConversion
  Position Command : Subsystem
  mapping : Subsystem
  FMS_Out : Outport
  wires:
  Constant2/1 -> Data Type Conversion3/1
  Constant5/1 -> Data Type Conversion1/1
  Constant1/1 -> Data Type Conversion2/1
  Data Type Conversion3/1 -> Bus Assignment/4
  Data Type Conversion2/1 -> Bus Assignment/3
  Bus Assignment/1 -> FMS_Out/1
  Data Type Conversion1/1 -> Bus Assignment/2
  Constant/1 -> Bus Assignment/1
  FMS_In/1 -> mapping/1(FMS_In), Position Command/1(FMS_In)
  Position Command/1(ay_cmd_mPs2) -> Bus Assignment/9
  Constant3/1 -> Bus Assignment/5
  mapping/1(v_cmd) -> Bus Assignment/6
  mapping/2(w_cmd) -> Bus Assignment/7
  mapping/3(psi_rate_cmd) -> Bus Assignment/8

== system FMS/FMS Commander/Commander/Arm/FW_Mode ==
  In Bus Element{,1..2,6..7} (5 alike) : Inport  PortName=FMS_In
  Action Port : ActionPort  InitializeStates=reset  ActionType=case
  Assist : Subsystem  TreatAsAtomicUnit=on
  Auto : Subsystem  TreatAsAtomicUnit=on
  Bus Selector : BusSelector  OutputSignals=vehicle_state
  Manual : Subsystem  TreatAsAtomicUnit=on
  Merge : Merge  Inputs=5
  SubMode : Subsystem  TreatAsAtomicUnit=on
  Switch Case : SwitchCase  CaseConditions={[VehicleState.Land,VehicleState.Return,VehicleState.Takeoff,VehicleState.Hold], [VehicleState.Offboard,VehicleState.Mission],[VehicleState.Acro,VehicleState.Stabilize,VehicleState.Altitude,VehicleState.Position],VehicleState.Manual}
  Unknown : Subsystem  TreatAsAtomicUnit=on
  FMS_Out : Outport
  wires:
  Merge/1 -> FMS_Out/1
  Switch Case/1 -> SubMode/Action
  Switch Case/2 -> Auto/Action
  Switch Case/3 -> Assist/Action
  Switch Case/4 -> Manual/Action
  SubMode/1(FMS_Out) -> Merge/1
  Auto/1(FMS_Out) -> Merge/2
  Assist/1(FMS_Out) -> Merge/3
  Manual/1(FMS_Out) -> Merge/4
  In Bus Element/1 -> SubMode/1(FMS_In)
  In Bus Element1/1 -> Assist/1(FMS_In)
  In Bus Element6/1 -> Auto/1(FMS_In)
  In Bus Element7/1 -> Manual/1(FMS_In)
  Switch Case/5 -> Unknown/Action
  Unknown/1(FMS_Out) -> Merge/5
  In Bus Element2/1 -> Bus Selector/1
  Bus Selector/1 -> Switch Case/1  "<vehicle_state>"

== system FMS/FMS Commander/Commander/Arm/MC_Mode ==
  In Bus Element{,1..2,6..7} (5 alike) : Inport  PortName=FMS_In
  Action Port : ActionPort  InitializeStates=reset  ActionType=default
  Assist : Subsystem  TreatAsAtomicUnit=on
  Auto : Subsystem  TreatAsAtomicUnit=on
  Bus Selector : BusSelector  OutputSignals=vehicle_state
  Manual : Subsystem  TreatAsAtomicUnit=on
  Merge : Merge  Inputs=5
  SubMode : Subsystem  TreatAsAtomicUnit=on
  Switch Case : SwitchCase  CaseConditions={[VehicleState.Land,VehicleState.Return,VehicleState.Takeoff,VehicleState.Hold], [VehicleState.Offboard,VehicleState.Mission],[VehicleState.Acro,VehicleState.Stabilize,VehicleState.Altitude,VehicleState.Position],VehicleState.Manual}
  Unknown : Subsystem  TreatAsAtomicUnit=on
  FMS_Out : Outport
  wires:
  Merge/1 -> FMS_Out/1
  Switch Case/1 -> SubMode/Action
  Switch Case/2 -> Auto/Action
  Switch Case/3 -> Assist/Action
  Switch Case/4 -> Manual/Action
  SubMode/1(FMS_Out) -> Merge/1
  Auto/1(FMS_Out) -> Merge/2
  Assist/1(FMS_Out) -> Merge/3
  Manual/1(FMS_Out) -> Merge/4
  In Bus Element/1 -> SubMode/1(FMS_In)
  In Bus Element1/1 -> Assist/1(FMS_In)
  In Bus Element6/1 -> Auto/1(FMS_In)
  In Bus Element7/1 -> Manual/1(FMS_In)
  Switch Case/5 -> Unknown/Action
  Unknown/1(FMS_Out) -> Merge/5
  In Bus Element2/1 -> Bus Selector/1
  Bus Selector/1 -> Switch Case/1  "<vehicle_state>"

== system FMS/FMS Commander/Commander/Bus_Constructor/timestamp ==
  Constant : Constant  Value=sample_time
  Data Type Conversion : DataTypeConversion  OutDataTypeStr=uint32
  Discrete-Time Integrator : DiscreteIntegrator  IntegratorMethod=Accumulation: Forward Euler  SampleTime=-1  ICPrevOutput=DiscIntNeverNeededParam  ICPrevScaledInput=DiscIntNeverNeededParam
  timestamp_ms : Outport
  wires:
  Discrete-Time Integrator/1 -> Data Type Conversion/1
  Constant/1 -> Discrete-Time Integrator/1
  Data Type Conversion/1 -> timestamp_ms/1

== system FMS/FMS Commander/Commander/Arm/BackwardTrans_Mode/Position Command ==
  FMS_In : Inport
  Controller : Subsystem
  Detect Movement : Subsystem
  ay_cmd_mPs2 : Outport
  wires:
  FMS_In/1 -> Controller/2(FMS_In), Detect Movement/1(FMS_In)
  Controller/1(ay_cmd_mPs2) -> ay_cmd_mPs2/1
  Detect Movement/1(motion_state) -> Controller/1(motion_state)

== system FMS/FMS Commander/Commander/Arm/BackwardTrans_Mode/mapping ==
  FMS_In : Inport
  Bus Selector : BusSelector  OutputSignals=Pilot_Cmd.stick_roll,Pilot_Cmd.stick_pitch,Pilot_Cmd.stick_yaw
  DeadZone : Subsystem  mask{th=FMS_PARAM.THROTTLE_DZ}
      mask prompts: th "Threshold"
      mask Display: disp('Dead Zone')
  DeadZone1 : Subsystem  mask{th=FMS_PARAM.ROLL_DZ}
      mask prompts: th "Threshold"
      mask Display: disp('Dead Zone')
  DeadZone2 : Subsystem  mask{th=FMS_PARAM.YAW_DZ}
      mask prompts: th "Threshold"
      mask Display: disp('Dead Zone')
  Gain1 : Gain  Gain=-FMS_PARAM.VEL_Z_LIM/2  OutDataTypeStr=single
  Gain2 : Gain  Gain=FMS_PARAM.YAW_RATE_LIM/2  OutDataTypeStr=single
  Gain6 : Gain  Gain=FMS_PARAM.VEL_XY_LIM/2  OutDataTypeStr=single
  TD : Subsystem
  TD1 : Subsystem
  TD2 : Subsystem
  v_cmd : Outport
  w_cmd : Outport  Port=2
  psi_rate_cmd : Outport  Port=3
  wires:
  FMS_In/1 -> Bus Selector/1
  Bus Selector/1 -> DeadZone1/1(u)  "<stick_roll>"
  DeadZone1/1(y) -> Gain6/1
  Bus Selector/2 -> DeadZone/1(u)  "<stick_pitch>"
  Gain1/1 -> TD2/1(v)
  Bus Selector/3 -> DeadZone2/1(u)  "<stick_yaw>"
  Gain2/1 -> TD1/1(v)
  DeadZone/1(y) -> Gain1/1
  DeadZone2/1(y) -> Gain2/1
  Gain6/1 -> TD/1(v)
  TD/1(v1) -> v_cmd/1
  TD1/1(v1) -> psi_rate_cmd/1
  TD2/1(v1) -> w_cmd/1

== system FMS/FMS Commander/Commander/Arm/FW_Mode/Assist ==
  In Bus Element{1..3,5} (4 alike) : Inport  PortName=FMS_In
  Action Port : ActionPort  InitializeStates=reset  ActionType=case
  Altitude : Subsystem
      settings: UndoDeleteFcn=Stateflow.SLINSF.SimulinkMan.restorePreDeleteFcn  PreDeleteFcn=Stateflow.SLINSF.SimulinkMan.removePreDeleteFcn
  Bus Selector : BusSelector  OutputSignals=vehicle_state
  Merge : Merge  Inputs=4
  Position : Subsystem
      settings: UndoDeleteFcn=Stateflow.SLINSF.SimulinkMan.restorePreDeleteFcn  PreDeleteFcn=Stateflow.SLINSF.SimulinkMan.removePreDeleteFcn
  Stabilize : Subsystem
      settings: UndoDeleteFcn=Stateflow.SLINSF.SimulinkMan.restorePreDeleteFcn  PreDeleteFcn=Stateflow.SLINSF.SimulinkMan.removePreDeleteFcn
  Switch Case : SwitchCase  CaseConditions={VehicleState.Stabilize,VehicleState.Altitude,VehicleState.Position}
  Unknown : Subsystem  TreatAsAtomicUnit=on
  FMS_Out : Outport
  wires:
  In Bus Element1/1 -> Position/1(FMS_In)
  In Bus Element2/1 -> Altitude/1(FMS_In)
  In Bus Element3/1 -> Stabilize/1(FMS_In)
  Merge/1 -> FMS_Out/1
  In Bus Element5/1 -> Bus Selector/1
  Bus Selector/1 -> Switch Case/1  "<vehicle_state>"
  Stabilize/1(FMS_Out) -> Merge/1
  Altitude/1(FMS_Out) -> Merge/2
  Position/1(FMS_Out) -> Merge/3
  Unknown/1(FMS_Out) -> Merge/4
  Switch Case/4 -> Unknown/Action
  Switch Case/1 -> Stabilize/Action
  Switch Case/2 -> Altitude/Action
  Switch Case/3 -> Position/Action

== system FMS/FMS Commander/Commander/Arm/FW_Mode/Auto ==
  In Bus Element6 : Inport  PortName=FMS_In
  In Bus Element1 : Inport  PortName=FMS_In
  In Bus Element2 : Inport  PortName=FMS_In
  Action Port : ActionPort  InitializeStates=reset  ActionType=case
  Bus Selector : BusSelector  OutputSignals=vehicle_state
  Merge : Merge  Inputs=3
  Mission : Subsystem
      settings: UndoDeleteFcn=Stateflow.SLINSF.SimulinkMan.restorePreDeleteFcn  PreDeleteFcn=Stateflow.SLINSF.SimulinkMan.removePreDeleteFcn
  Offboard : Subsystem
      settings: UndoDeleteFcn=Stateflow.SLINSF.SimulinkMan.restorePreDeleteFcn  PreDeleteFcn=Stateflow.SLINSF.SimulinkMan.removePreDeleteFcn
  Switch Case : SwitchCase  CaseConditions={VehicleState.Offboard,VehicleState.Mission}
  Unknown : Subsystem  TreatAsAtomicUnit=on
  FMS_Out : Outport
  wires:
  Merge/1 -> FMS_Out/1
  In Bus Element6/1 -> Offboard/1(FMS_In)
  Switch Case/1 -> Offboard/Action
  In Bus Element1/1 -> Mission/1(FMS_In)
  Switch Case/2 -> Mission/Action
  Offboard/1(FMS_Out) -> Merge/1
  Mission/1(FMS_Out) -> Merge/2
  Unknown/1(FMS_Out) -> Merge/3
  Switch Case/3 -> Unknown/Action
  In Bus Element2/1 -> Bus Selector/1
  Bus Selector/1 -> Switch Case/1  "<vehicle_state>"

== system FMS/FMS Commander/Commander/Arm/FW_Mode/Manual ==
  In Bus Element7 : Inport  PortName=FMS_In
  Action Port : ActionPort  InitializeStates=reset  ActionType=case
  Bus Assignment : BusAssignment  AssignedSignals=reset,status,state,ctrl_mode,p_cmd,q_cmd,r_cmd,u_cmd
  Bus Selector : BusSelector  OutputSignals=Pilot_Cmd.stick_roll,Pilot_Cmd.stick_pitch,Pilot_Cmd.stick_yaw,Pilot_Cmd.stick_throttle
  Constant : Constant  Value=0  OutDataTypeStr=Bus: FMS_Out_Bus
  Constant1 : Constant  Value=VehicleStatus.Arm
  Constant2 : Constant  OutDataTypeStr=Inherit: Inherit via back propagation
  Constant3 : Constant  Value=ControlMode.Manual
  Constant5 : Constant  Value=VehicleState.Manual
  Data Type Conversion : DataTypeConversion
  Data Type Conversion1 : DataTypeConversion
  Data Type Conversion2 : DataTypeConversion
  DeadZone : Subsystem  mask{th=FMS_PARAM.ROLL_DZ}
      mask prompts: th "Threshold"
      mask Display: disp('Dead Zone')
  DeadZone1 : Subsystem  mask{th=FMS_PARAM.PITCH_DZ}
      mask prompts: th "Threshold"
      mask Display: disp('Dead Zone')
  DeadZone2 : Subsystem  mask{th=FMS_PARAM.YAW_DZ}
      mask prompts: th "Threshold"
      mask Display: disp('Dead Zone')
  DeadZone3 : Subsystem  mask{th=FMS_PARAM.THROTTLE_DZ}
      mask prompts: th "Threshold"
      mask Display: disp('Dead Zone')
  Gain : Gain  Gain=-1
  FMS_Out : Outport
  wires:
  Data Type Conversion1/1 -> Bus Assignment/4
  Data Type Conversion/1 -> Bus Assignment/3
  Constant5/1 -> Data Type Conversion1/1
  Constant/1 -> Bus Assignment/1
  Bus Assignment/1 -> FMS_Out/1
  Constant2/1 -> Bus Assignment/2
  Constant1/1 -> Data Type Conversion/1
  In Bus Element7/1 -> Bus Selector/1
  Bus Selector/1 -> DeadZone/1(u)  "<stick_roll>"
  Constant3/1 -> Data Type Conversion2/1
  Data Type Conversion2/1 -> Bus Assignment/5
  Bus Selector/2 -> DeadZone1/1(u)  "<stick_pitch>"
  Bus Selector/3 -> DeadZone2/1(u)  "<stick_yaw>"
  Bus Selector/4 -> DeadZone3/1(u)  "<stick_throttle>"
  DeadZone/1(y) -> Bus Assignment/6
  DeadZone1/1(y) -> Gain/1
  Gain/1 -> Bus Assignment/7
  DeadZone2/1(y) -> Bus Assignment/8
  DeadZone3/1(y) -> Bus Assignment/9
